simulink model "simulink_flightgear_control_trim_wind_5"  (R2023a)
settings: Solver=VariableStepAuto  StartTime=0  StopTime=inf  FixedStep=0.1  RelTol=1e-3
values from neighbouring files (symbols this model uses):
  alpha = -5:0.1:25    [Boeing747model.m]
  alpha1 = 0:0.1:14    [Boeing747model.m]
  alpha2 = -5:0.1:25    [Boeing747model.m]
  alpha3 = -5:0.1:17    [Boeing747model.m]
  beta = -15:0.1:15    [Boeing747model.m]
  CL = 0:0.01:1.4    [Boeing747model.m]
  da = 0:1:20    [Boeing747model.m]
  dr = [0 5 10 15 20 25]    [Boeing747model.m]
  EPR_ = 0:0.1:1.8    [Boeing747model.m]    (also in engine.m)
  flap = [0 10 20 25 30]    [Boeing747model.m]
  high1 = 0:10000:40000    [Boeing747model.m]
  high2 = 0:20000:40000    [Boeing747model.m]
  high3 = [0 15000 25000 35000 40000]    [Boeing747model.m]    (also in engine.m)
  high4 = [0 10000 20000 40000]    [Boeing747model.m]
  interp_result = table2array(resultTable(:,2:end))    [Boeing747model.m]
  interp_result_mach = 0:0.1:0.9    [Boeing747model.m]
  interp_result_N1 = 80:5:110    [Boeing747model.m]
  m2ft = 3.280839895013    (= 3.28083989501)    [Boeing747model.m]    (also in engine.m)
  mach = 0:0.02:0.9    [Boeing747model.m]    (also in engine.m)
  mach1 = [0 0.3 0.5 0.7 0.8 0.84 0.86 0.88 0.9]    [Boeing747model.m]
  mach2 = [0 0.3 0.5 0.7 0.8 0.9]    [Boeing747model.m]
  mach3 = [0 0.1 0.3 0.5 0.6 0.7 0.8 0.9]    [Boeing747model.m]    (also in engine.m = [0 0.1 0.3 0.5  0.7 0.8 0.9])
  mach5 = [0 0.6 0.8 0.85 0.9]    [Boeing747model.m]
  mach6 = [0 0.6 0.8 0.9]    [Boeing747model.m]
  mach7 = [0 0.3 0.5 0.74 0.8 0.84 0.86 0.88 0.9]    [Boeing747model.m]
  mach8 = [0 0.3 0.5 0.74 0.8 0.84 0.86 0.88 0.9]    [Boeing747model.m]
  model = 'simulink_flightgear_control_trim_wind_5'    [traimcode.m]
  ms2kts = 1.943844492609    (= 1.94384449261)    [Boeing747model.m]    (also in engine.m)
  powerangle_ = 0:1:130    [Boeing747model.m]    (also in engine.m)
  T = [-45 0 60 120]    [Boeing747model.m]    (also in engine.m)
  V_E = 0:20:250    [Boeing747model.m]
undefined symbols (not defined in the file or in its folder): Earth, F, ft, Light, m, MIL, Model, Newton, P3DAERO, Raphson, Receive, s, Send, Unit, WGS84, Wind
libraries: simulink_extras x115, aerolibconvert2 x16, simulink x4, aerolibfltsims x3, shared6dof x1, aerolibasang x1, aerolibtransform2 x1, aerolibatmos2 x1, aerolibobsolete x1, aerolibwind2 x1
(part 4 of 5)

== system simulink_flightgear_control_trim_wind_5/Plane/气动系数/Subsystem58/Subsystem41 ==
  In1 : Inport
  In2 : Inport  Port=2
  Radians in : Inport  Port=3
  Radians in1 : Inport  Port=4
  1-D Lookup Table79 : Lookup_n-D  NumberOfTableDimensions=1  BreakpointsForDimension1=P3DAERO.delata_CN_RL_25(1,:)  Table=P3DAERO.delata_CN_RL_25(2,:)  InternalRulePriority=Speed  RndMeth=Simplest
  1-D Lookup Table81 : Lookup_n-D  NumberOfTableDimensions=1  BreakpointsForDimension1=P3DAERO.k_delta_RL(1,:)  Table=P3DAERO.k_delta_RL(2,:)  InternalRulePriority=Speed  RndMeth=Simplest
  2-D Lookup Table15 : Lookup_n-D  BreakpointsForDimension1=high1  BreakpointsForDimension2=mach  Table=P3DAERO.delata_CN_RL_25_mach  InternalRulePriority=Speed  RndMeth=Simplest
      settings: InputPortMap=u0,u1
  Abs5 : Abs  SaturateOnIntegerOverflow=off
  Constant34 : Constant
  Constant35 : Constant  Value=-1
  Gain10 : Gain  Gain=m2ft
  Product8 : Product  Inputs=4
  Radians to Degrees22 : simulink_extras/Transformations/Radians to Degrees
  Radians to Degrees23 : simulink_extras/Transformations/Radians to Degrees
  Switch6 : Switch  SaturateOnIntegerOverflow=off  InputSameDT=off
  Out1 : Outport
  wires:
  2-D Lookup Table15/1 -> Product8/1
  Constant35/1 -> Switch6/3
  Constant34/1 -> Switch6/1
  1-D Lookup Table81/1 -> Product8/3
  Radians in1/1 -> Switch6/2, Radians to Degrees23/1
  Radians to Degrees22/1 -> 1-D Lookup Table79/1
  Abs5/1 -> 1-D Lookup Table81/1
  Gain10/1 -> 2-D Lookup Table15/1
  Switch6/1 -> Product8/4
  Radians to Degrees23/1 -> Abs5/1
  1-D Lookup Table79/1 -> Product8/2
  In2/1 -> 2-D Lookup Table15/2
  In1/1 -> Gain10/1
  Product8/1 -> Out1/1
  Radians in/1 -> Radians to Degrees22/1

== system simulink_flightgear_control_trim_wind_5/Plane/气动系数/Subsystem58/Subsystem42 ==
  note: 速度ft/s
  note: beta角速度
  Radians in : Inport
  In2 : Inport  Port=2
  In3 : Inport  Port=3
  In4 : Inport  Port=4
  In5 : Inport  Port=5
  1-D Lookup Table2 : Lookup_n-D  NumberOfTableDimensions=1  BreakpointsForDimension1=P3DAERO.dot_CN_dot_beta_dian(1,:)  Table=P3DAERO.dot_CN_dot_beta_dian(2,:)  InternalRulePriority=Speed  RndMeth=Simplest
  2-D Lookup Table4 : Lookup_n-D  BreakpointsForDimension1=high1  BreakpointsForDimension2=mach  Table=P3DAERO.dot_CN_dot_beta_dian_mach  InternalRulePriority=Speed  RndMeth=Simplest
      settings: InputPortMap=u0,u1
  Constant7 : Constant  Value=2
  Constant8 : Constant  Value=195.7
  Divide2 : Product  Inputs=**//
  Gain : Gain  Gain=-1
  Gain5 : Gain  Gain=m2ft
  Product2 : Product  Inputs=3
  Radians to Degrees : simulink_extras/Transformations/Radians to Degrees
  Scope1 : Scope
  Out1 : Outport
  wires:
  2-D Lookup Table4/1 -> Product2/2
  Divide2/1 -> Product2/3
  1-D Lookup Table2/1 -> Product2/1
  In3/1 -> 2-D Lookup Table4/2
  Constant8/1 -> Divide2/2
  Gain5/1 -> 2-D Lookup Table4/1
  Radians to Degrees/1 -> 1-D Lookup Table2/1
  Constant7/1 -> Divide2/4
  Radians in/1 -> Radians to Degrees/1
  In2/1 -> Gain5/1
  In4/1 -> Divide2/1
  Product2/1 -> Gain/1
  In5/1 -> Divide2/3
  Gain/1 -> Scope1/1, Out1/1

== system simulink_flightgear_control_trim_wind_5/Plane/气动系数/Subsystem58/Subsystem43 ==
  note: 滚转角速度
  In1 : Inport
  In2 : Inport  Port=2
  Radians in : Inport  Port=3
  In4 : Inport  Port=4
  In5 : Inport  Port=5
  2-D Lookup Table5 : Lookup_n-D  BreakpointsForDimension1=flap  BreakpointsForDimension2=alpha  Table=P3DAERO.dot_CN_dot_p  InternalRulePriority=Speed  RndMeth=Simplest
      settings: InputPortMap=u0,u1
  2-D Lookup Table6 : Lookup_n-D  BreakpointsForDimension1=mach5  BreakpointsForDimension2=alpha  Table=P3DAERO.dot_CN_dot_p_mach  InternalRulePriority=Speed  RndMeth=Simplest
      settings: InputPortMap=u0,u1
  Constant24 : Constant  Value=2
  Constant25 : Constant  Value=195.7
  Divide3 : Product  Inputs=**//
  Divide4 : Product  Inputs=**
  Gain5 : Gain  Gain=-1
  Radians to Degrees3 : simulink_extras/Transformations/Radians to Degrees
  Radians to Degrees5 : simulink_extras/Transformations/Radians to Degrees
  Scope : Scope
  Switch11 : Switch  Criteria=u2 ~= 0  Threshold=0.6  SaturateOnIntegerOverflow=off  InputSameDT=off
  Out1 : Outport
  wires:
  In2/1 -> Switch11/2, 2-D Lookup Table5/1
  Divide4/1 -> Gain5/1
  Switch11/1 -> Divide4/2
  2-D Lookup Table6/1 -> Switch11/3
  2-D Lookup Table5/1 -> Switch11/1
  Radians to Degrees5/1 -> 2-D Lookup Table5/2
  Radians in/1 -> Radians to Degrees3/1, Radians to Degrees5/1
  Radians to Degrees3/1 -> 2-D Lookup Table6/2
  Constant25/1 -> Divide3/2
  In4/1 -> 2-D Lookup Table6/1
  Divide3/1 -> Divide4/1
  Constant24/1 -> Divide3/4
  In1/1 -> Divide3/1
  In5/1 -> Divide3/3
  Gain5/1 -> Scope/1, Out1/1

== system simulink_flightgear_control_trim_wind_5/Plane/气动系数/Subsystem58/Subsystem44 ==
  u : Inport
  In2 : Inport  Port=2
  Radians in : Inport  Port=3
  In4 : Inport  Port=4
  In5 : Inport  Port=5
  In6 : Inport  Port=6
  In7 : Inport  Port=7
  2-D Lookup Table7 : Lookup_n-D  BreakpointsForDimension1=flap  BreakpointsForDimension2=alpha  Table=P3DAERO.dot_CN_dot_r25  InternalRulePriority=Speed  RndMeth=Simplest
      settings: InputPortMap=u0,u1
  2-D Lookup Table8 : Lookup_n-D  BreakpointsForDimension1=high1  BreakpointsForDimension2=mach  Table=P3DAERO.dot_CN_dot_r_mach  InternalRulePriority=Speed  RndMeth=Simplest
      settings: InputPortMap=u0,u1
  Constant13 : Constant  Value=2
  Constant14 : Constant  Value=195.7
  Divide6 : Product  Inputs=**//
  Gain7 : Gain  Gain=m2ft
  MATLAB Function2 : MATLAB Function  TreatAsAtomicUnit=on
  MATLAB Function3 : MATLAB Function  Commented=on  TreatAsAtomicUnit=on
  Product1 : Product  Inputs=4
  Radians to Degrees2 : simulink_extras/Transformations/Radians to Degrees
  Scope : Scope
  Scope1 : Scope
  Out1 : Outport
  wires:
  Constant13/1 -> Divide6/4
  2-D Lookup Table7/1 -> Product1/2
  Radians to Degrees2/1 -> 2-D Lookup Table7/2
  MATLAB Function2/1(y) -> Scope1/1, Product1/1
  2-D Lookup Table8/1 -> Product1/3
  Constant14/1 -> Divide6/2
  Gain7/1 -> 2-D Lookup Table8/1
  In2/1 -> 2-D Lookup Table7/1
  Radians in/1 -> Radians to Degrees2/1
  Divide6/1 -> Product1/4
  In5/1 -> 2-D Lookup Table8/2
  In4/1 -> Gain7/1
  In6/1 -> Divide6/1
  u/1 -> MATLAB Function2/1(u)
  In7/1 -> Divide6/3
  Product1/1 -> Scope/1, Out1/1

== system simulink_flightgear_control_trim_wind_5/Plane/气动系数/Subsystem58/Subsystem45 ==
  note: n地效修正
  In1 : Inport
  In2 : Inport  Port=2
  Radians in : Inport  Port=3
  1-D Lookup Table86 : Lookup_n-D  NumberOfTableDimensions=1  BreakpointsForDimension1=P3DAERO.k_ge(1,:)  Table=P3DAERO.k_ge(2,:)  InternalRulePriority=Speed  RndMeth=Simplest
  2-D Lookup Table9 : Lookup_n-D  BreakpointsForDimension1=flap  BreakpointsForDimension2=alpha1  Table=P3DAERO.Fn  InternalRulePriority=Speed  RndMeth=Simplest
      settings: InputPortMap=u0,u1
  Constant27 : Constant
  Gain3 : Gain  Gain=m2ft
  Product6 : Product
  Radians to Degrees7 : simulink_extras/Transformations/Radians to Degrees
  Saturation2 : Saturate  UpperLimit=14  LowerLimit=0
  Scope2 : Scope
  Sum19 : Sum
  Switch1 : Switch  Criteria=u2 > Threshold  Threshold=24  SaturateOnIntegerOverflow=off  InputSameDT=off
  Out1 : Outport
  wires:
  In2/1 -> 2-D Lookup Table9/1
  2-D Lookup Table9/1 -> Product6/2
  Gain3/1 -> 1-D Lookup Table86/1
  Radians to Degrees7/1 -> Saturation2/1
  Sum19/1 -> Switch1/3
  Saturation2/1 -> 2-D Lookup Table9/2
  1-D Lookup Table86/1 -> Product6/1, Scope2/1
  Constant27/1 -> Sum19/1, Switch1/1
  Product6/1 -> Sum19/2
  Radians in/1 -> Radians to Degrees7/1
  Switch1/1 -> Out1/1
  In1/1 -> Switch1/2, Gain3/1

== system simulink_flightgear_control_trim_wind_5/Plane/气动系数/Subsystem58/Subsystem46 ==
  In1 : Inport
  In2 : Inport  Port=2
  Radians in : Inport  Port=3
  In4 : Inport  Port=4
  Radians in1 : Inport  Port=5
  1-D Lookup Table1 : Lookup_n-D  BreakpointsForDimension1=flap  BreakpointsForDimension2=alpha  Table=P3DAERO.delta_CN_ai  InternalRulePriority=Speed  RndMeth=Simplest
      settings: InputPortMap=u0,u1
  1-D Lookup Table3 : Lookup_n-D  BreakpointsForDimension1=flap  BreakpointsForDimension2=da  Table=P3DAERO.k_delta_ai  InternalRulePriority=Speed  RndMeth=Simplest
      settings: InputPortMap=u0,u1
  1-D Lookup Table54 : Lookup_n-D  NumberOfTableDimensions=1  BreakpointsForDimension1=P3DAERO.delta_CN_ai_mach(1,:)  Table=P3DAERO.delta_CN_ai_mach(2,:)  InternalRulePriority=Speed  RndMeth=Simplest
  Constant16 : Constant
  Constant18 : Constant  Value=-1
  Constant20 : Constant  Value=2
  Product4 : Product  Inputs=3
  Product5 : Product  Inputs=4
  Radians to Degrees8 : simulink_extras/Transformations/Radians to Degrees
  Radians to Degrees9 : simulink_extras/Transformations/Radians to Degrees
  Scope4 : Scope
  Switch2 : Switch  SaturateOnIntegerOverflow=off  InputSameDT=off
  Out1 : Outport
  wires:
  1-D Lookup Table3/1 -> Product5/4
  Constant18/1 -> Switch2/3
  1-D Lookup Table54/1 -> Product5/1
  Radians to Degrees8/1 -> 1-D Lookup Table3/2
  Switch2/1 -> Product4/3
  1-D Lookup Table1/1 -> Product5/2
  Radians to Degrees9/1 -> 1-D Lookup Table1/2
  Radians in1/1 -> Switch2/2, Radians to Degrees8/1
  Constant16/1 -> Switch2/1
  Constant20/1 -> Product4/1
  Product5/1 -> Product4/2, Scope4/1
  In2/1 -> 1-D Lookup Table3/1, 1-D Lookup Table1/1
  In4/1 -> Product5/3
  Radians in/1 -> Radians to Degrees9/1
  Product4/1 -> Out1/1
  In1/1 -> 1-D Lookup Table54/1

== system simulink_flightgear_control_trim_wind_5/Plane/气动系数/Subsystem58/Subsystem47 ==
  note: 15down
  note: 25up
  In1 : Inport
  Radians in : Inport  Port=2
  In3 : Inport  Port=3
  Radians in1 : Inport  Port=4
  1-D Lookup Table60 : Lookup_n-D  NumberOfTableDimensions=1  BreakpointsForDimension1=P3DAERO.k_delata_Ao_down(1,:)  Table=P3DAERO.k_delata_Ao_down(2,:)  InternalRulePriority=Speed  RndMeth=Simplest
  1-D Lookup Table61 : Lookup_n-D  NumberOfTableDimensions=1  BreakpointsForDimension1=P3DAERO.k_delata_Ao_up(1,:)  Table=P3DAERO.k_delata_Ao_up(2,:)  InternalRulePriority=Speed  RndMeth=Simplest
  2-D Lookup Table10 : Lookup_n-D  BreakpointsForDimension1=flap  BreakpointsForDimension2=alpha  Table=P3DAERO.delata_CN_Ao_15down  InternalRulePriority=Speed  RndMeth=Simplest
      settings: InputPortMap=u0,u1
  2-D Lookup Table11 : Lookup_n-D  BreakpointsForDimension1=flap  BreakpointsForDimension2=alpha  Table=P3DAERO.delata_CN_Ao_25up  InternalRulePriority=Speed  RndMeth=Simplest
      settings: InputPortMap=u0,u1
  Abs3 : Abs  SaturateOnIntegerOverflow=off
  Abs4 : Abs  SaturateOnIntegerOverflow=off
  Product13 : Product  Inputs=3
  Radians to Degrees{10,15..17} (4 alike) : simulink_extras/Transformations/Radians to Degrees
  Scope34 : Scope
  Scope37 : Scope
  Scope38 : Scope
  Switch7 : Switch  SaturateOnIntegerOverflow=off  InputSameDT=off
  Switch8 : Switch  SaturateOnIntegerOverflow=off  InputSameDT=off
  Out1 : Outport
  wires:
  Switch7/1 -> Product13/2, Scope34/1
  Radians to Degrees16/1 -> 2-D Lookup Table11/2
  Radians in/1 -> Radians to Degrees17/1, Switch8/2, Radians to Degrees15/1, Switch7/2
  2-D Lookup Table11/1 -> Switch8/3
  Abs3/1 -> 1-D Lookup Table60/1
  Switch8/1 -> Product13/3, Scope37/1
  Radians to Degrees15/1 -> Abs3/1
  In3/1 -> 2-D Lookup Table11/1, 2-D Lookup Table10/1
  1-D Lookup Table60/1 -> Switch7/1
  2-D Lookup Table10/1 -> Switch8/1
  Radians to Degrees10/1 -> 2-D Lookup Table10/2
  Abs4/1 -> 1-D Lookup Table61/1
  Radians to Degrees17/1 -> Abs4/1
  1-D Lookup Table61/1 -> Switch7/3
  Product13/1 -> Out1/1, Scope38/1
  Radians in1/1 -> Radians to Degrees16/1, Radians to Degrees10/1
  In1/1 -> Product13/1

== system simulink_flightgear_control_trim_wind_5/Plane/气动系数/Subsystem58/Subsystem48 ==
  note: 15down
  note: 25up
  In1 : Inport
  Radians in : Inport  Port=2
  In3 : Inport  Port=3
  Radians in1 : Inport  Port=4
  1-D Lookup Table72 : Lookup_n-D  NumberOfTableDimensions=1  BreakpointsForDimension1=P3DAERO.k_delata_Ao_down(1,:)  Table=P3DAERO.k_delata_Ao_down(2,:)  InternalRulePriority=Speed  RndMeth=Simplest
  1-D Lookup Table73 : Lookup_n-D  NumberOfTableDimensions=1  BreakpointsForDimension1=P3DAERO.k_delata_Ao_up(1,:)  Table=P3DAERO.k_delata_Ao_up(2,:)  InternalRulePriority=Speed  RndMeth=Simplest
  2-D Lookup Table12 : Lookup_n-D  BreakpointsForDimension1=flap  BreakpointsForDimension2=alpha  Table=P3DAERO.delata_CN_Ao_15down  InternalRulePriority=Speed  RndMeth=Simplest
      settings: InputPortMap=u0,u1
  2-D Lookup Table13 : Lookup_n-D  BreakpointsForDimension1=flap  BreakpointsForDimension2=alpha  Table=P3DAERO.delata_CN_Ao_25up  InternalRulePriority=Speed  RndMeth=Simplest
      settings: InputPortMap=u0,u1
  Abs1 : Abs  SaturateOnIntegerOverflow=off
  Abs2 : Abs  SaturateOnIntegerOverflow=off
  Product14 : Product  Inputs=3
  Radians to Degrees{11..14} (4 alike) : simulink_extras/Transformations/Radians to Degrees
  Scope39 : Scope
  Scope43 : Scope
  Switch3 : Switch  SaturateOnIntegerOverflow=off  InputSameDT=off
  Switch9 : Switch  SaturateOnIntegerOverflow=off  InputSameDT=off
  Out1 : Outport
  wires:
  Switch3/1 -> Product14/3
  Radians to Degrees12/1 -> Abs1/1
  In3/1 -> 2-D Lookup Table13/1, 2-D Lookup Table12/1
  1-D Lookup Table72/1 -> Switch9/1
  Radians in1/1 -> Radians to Degrees14/1, Radians to Degrees11/1
  2-D Lookup Table13/1 -> Switch3/3
  Abs1/1 -> 1-D Lookup Table72/1
  Switch9/1 -> Product14/2, Scope39/1
  Radians to Degrees13/1 -> Abs2/1
  Radians to Degrees11/1 -> 2-D Lookup Table12/2
  Radians to Degrees14/1 -> 2-D Lookup Table13/2
  Product14/1 -> Out1/1, Scope43/1
  2-D Lookup Table12/1 -> Switch3/1
  Abs2/1 -> 1-D Lookup Table73/1
  1-D Lookup Table73/1 -> Switch9/3
  Radians in/1 -> Radians to Degrees13/1, Switch3/2, Radians to Degrees12/1, Switch9/2
  In1/1 -> Product14/1

== system simulink_flightgear_control_trim_wind_5/Plane/气动系数/Subsystem58/Subsystem49 ==
  note: Y beta地效修正
  In1 : Inport
  In2 : Inport  Port=2
  Radians in : Inport  Port=3
  1-D Lookup Table97 : Lookup_n-D  NumberOfTableDimensions=1  BreakpointsForDimension1=P3DAERO.k_ge(1,:)  Table=P3DAERO.k_ge(2,:)  InternalRulePriority=Speed  RndMeth=Simplest
  2-D Lookup Table2 : Lookup_n-D  BreakpointsForDimension1=flap  BreakpointsForDimension2=alpha1  Table=P3DAERO.Fc_beta  InternalRulePriority=Speed  RndMeth=Simplest
      settings: InputPortMap=u0,u1
  Constant : Constant  Value=4.58
  Constant21 : Constant
  Gain14 : Gain  Gain=m2ft
  Product16 : Product
  Radians to Degrees1 : simulink_extras/Transformations/Radians to Degrees
  Saturation2 : Saturate  UpperLimit=14  LowerLimit=0
  Scope31 : Scope
  Scope48 : Scope
  Sum : Sum  Inputs=|+-
  Sum11 : Sum
  Switch5 : Switch  Criteria=u2 > Threshold  Threshold=24  SaturateOnIntegerOverflow=off  InputSameDT=off
  Out1 : Outport
  wires:
  Gain14/1 -> 1-D Lookup Table97/1
  Switch5/1 -> Out1/1, Scope31/1
  Saturation2/1 -> 2-D Lookup Table2/2
  Radians to Degrees1/1 -> Saturation2/1
  Product16/1 -> Sum11/2
  Constant21/1 -> Sum11/1, Switch5/1
  1-D Lookup Table97/1 -> Scope48/1, Product16/1
  Sum11/1 -> Switch5/3
  2-D Lookup Table2/1 -> Product16/2
  In2/1 -> 2-D Lookup Table2/1
  Radians in/1 -> Radians to Degrees1/1
  Constant/1 -> Sum/2
  In1/1 -> Sum/1
  Sum/1 -> Switch5/2, Gain14/1

== system simulink_flightgear_control_trim_wind_5/Plane/气动系数/Subsystem58/Subsystem5 ==
  note: 迎角角速度rad/s
  note: 速度ft/s
  note: dot_CL_dot_alpha_dian
  note: 平均气动弦长ft
  In1 : Inport
  In2 : Inport  Port=2
  In3 : Inport  Port=3
  1-D Lookup Table1 : Lookup_n-D  NumberOfTableDimensions=1  BreakpointsForDimension1=mach  Table=P3DAERO.dot_CL_dot_alpha_dian  InternalRulePriority=Speed  RndMeth=Simplest
  Constant7 : Constant  Value=2
  Constant9 : Constant  Value=27.3
  Divide : Product  Inputs=**//
  Gain8 : Gain
  Product2 : Product
  Scope5 : Scope
  Scope8 : Scope
  Scope9 : Scope
  Out1 : Outport
  wires:
  In2/1 -> 1-D Lookup Table1/1
  Gain8/1 -> Out1/1, Scope9/1
  Constant9/1 -> Divide/2
  Constant7/1 -> Divide/4
  Product2/1 -> Gain8/1
  Divide/1 -> Product2/2, Scope5/1
  1-D Lookup Table1/1 -> Product2/1, Scope8/1
  In1/1 -> Divide/1
  In3/1 -> Divide/3

== system simulink_flightgear_control_trim_wind_5/Plane/气动系数/Subsystem58/Subsystem50 ==
  In1 : Inport
  Radians in : Inport  Port=2
  In3 : Inport  Port=3
  In4 : Inport  Port=4
  2-D Lookup Table : Lookup_n-D  BreakpointsForDimension1=flap  BreakpointsForDimension2=alpha  Table=P3DAERO.dot_CC_dot_beta  InternalRulePriority=Speed  RndMeth=Simplest
      settings: InputPortMap=u0,u1
  2-D Lookup Table1 : Lookup_n-D  BreakpointsForDimension1=high1  BreakpointsForDimension2=mach  Table=P3DAERO.dot_CC_dot_beta_mach  InternalRulePriority=Speed  RndMeth=Simplest
      settings: InputPortMap=u0,u1
  Gain3 : Gain  Gain=m2ft
  Product : Product
  Radians to Degrees4 : simulink_extras/Transformations/Radians to Degrees
  Out1 : Outport
  wires:
  2-D Lookup Table/1 -> Product/1
  Gain3/1 -> 2-D Lookup Table1/1
  Radians to Degrees4/1 -> 2-D Lookup Table/2
  2-D Lookup Table1/1 -> Product/2
  In3/1 -> Gain3/1
  In4/1 -> 2-D Lookup Table1/2
  Radians in/1 -> Radians to Degrees4/1
  In1/1 -> 2-D Lookup Table/1
  Product/1 -> Out1/1

== system simulink_flightgear_control_trim_wind_5/Plane/气动系数/Subsystem58/Subsystem51 ==
  note: 滚转角速度
  note: bft
  note: 速度ft/s
  In1 : Inport
  In2 : Inport  Port=2
  In3 : Inport  Port=3
  Radians in : Inport  Port=4
  In5 : Inport  Port=5
  2-D Lookup Table3 : Lookup_n-D  BreakpointsForDimension1=flap  BreakpointsForDimension2=alpha  Table=P3DAERO.dot_CC_dot_p  InternalRulePriority=Speed  RndMeth=Simplest
      settings: InputPortMap=u0,u1
  2-D Lookup Table4 : Lookup_n-D  BreakpointsForDimension1=mach6  BreakpointsForDimension2=alpha  Table=P3DAERO.dot_CC_dot_p_mach  InternalRulePriority=Speed  RndMeth=Simplest
      settings: InputPortMap=u0,u1
  Constant10 : Constant  Value=2
  Constant12 : Constant  Value=195.7
  Divide1 : Product  Inputs=**//
  Divide3 : Product  Inputs=**
  Gain : Gain  Gain=-1
  Radians to Degrees5 : simulink_extras/Transformations/Radians to Degrees
  Radians to Degrees6 : simulink_extras/Transformations/Radians to Degrees
  Scope : Scope
  Switch3 : Switch  Criteria=u2 ~= 0  Threshold=0.6  SaturateOnIntegerOverflow=off  InputSameDT=off
  Out1 : Outport
  wires:
  Radians in/1 -> Radians to Degrees5/1, Radians to Degrees6/1
  In2/1 -> 2-D Lookup Table4/1
  In1/1 -> Divide1/1
  Divide1/1 -> Divide3/1
  Switch3/1 -> Divide3/2
  Radians to Degrees6/1 -> 2-D Lookup Table3/2
  2-D Lookup Table3/1 -> Switch3/1
  Constant12/1 -> Divide1/2
  Radians to Degrees5/1 -> 2-D Lookup Table4/2
  In3/1 -> Switch3/2, 2-D Lookup Table3/1
  Constant10/1 -> Divide1/4
  2-D Lookup Table4/1 -> Switch3/3
  Divide3/1 -> Scope/1, Gain/1
  In5/1 -> Divide1/3
  Gain/1 -> Out1/1

== system simulink_flightgear_control_trim_wind_5/Plane/气动系数/Subsystem58/Subsystem52 ==
  note: 速度ft/s
  note: 偏航角速度
  In1 : Inport
  Radians in : Inport  Port=2
  In3 : Inport  Port=3
  In4 : Inport  Port=4
  In5 : Inport  Port=5
  In6 : Inport  Port=6
  2-D Lookup Table5 : Lookup_n-D  BreakpointsForDimension1=flap  BreakpointsForDimension2=alpha  Table=P3DAERO.dot_CC_dot_r  InternalRulePriority=Speed  RndMeth=Simplest
      settings: InputPortMap=u0,u1
  2-D Lookup Table6 : Lookup_n-D  BreakpointsForDimension1=high4  BreakpointsForDimension2=mach  Table=P3DAERO.dot_CC_dot_r_mach  InternalRulePriority=Speed  RndMeth=Simplest
      settings: InputPortMap=u0,u1
  Constant7 : Constant  Value=2
  Constant8 : Constant  Value=195.7
  Divide2 : Product  Inputs=**//
  Gain4 : Gain  Gain=m2ft
  Product2 : Product  Inputs=3
  Radians to Degrees7 : simulink_extras/Transformations/Radians to Degrees
  Scope : Scope
  Out1 : Outport
  wires:
  2-D Lookup Table5/1 -> Product2/1
  In4/1 -> 2-D Lookup Table6/2
  Divide2/1 -> Product2/3
  Gain4/1 -> 2-D Lookup Table6/1
  Constant8/1 -> Divide2/2
  Radians to Degrees7/1 -> 2-D Lookup Table5/2
  2-D Lookup Table6/1 -> Product2/2
  Constant7/1 -> Divide2/4
  Radians in/1 -> Radians to Degrees7/1
  In1/1 -> 2-D Lookup Table5/1
  In3/1 -> Gain4/1
  In5/1 -> Divide2/1
  In6/1 -> Divide2/3
  Product2/1 -> Out1/1, Scope/1

== system simulink_flightgear_control_trim_wind_5/Plane/气动系数/Subsystem58/Subsystem53 ==
  In1 : Inport
  In2 : Inport  Port=2
  Radians in : Inport  Port=3
  Radians in1 : Inport  Port=4
  1-D Lookup Table101 : Lookup_n-D  NumberOfTableDimensions=1  BreakpointsForDimension1=P3DAERO.delta_CC_25_RU(1,:)  Table=P3DAERO.delta_CC_25_RU(2,:)  InternalRulePriority=Speed  RndMeth=Simplest
  1-D Lookup Table102 : Lookup_n-D  NumberOfTableDimensions=1  BreakpointsForDimension1=P3DAERO.k_delta_RU(1,:)  Table=P3DAERO.k_delta_RU(2,:)  InternalRulePriority=Speed  RndMeth=Simplest
  2-D Lookup Table7 : Lookup_n-D  BreakpointsForDimension1=high1  BreakpointsForDimension2=mach  Table=P3DAERO.delta_CC_25_RU_mach  InternalRulePriority=Speed  RndMeth=Simplest
      settings: InputPortMap=u0,u1
  Abs : Abs  SaturateOnIntegerOverflow=off
  Constant32 : Constant
  Constant33 : Constant  Value=-1
  Gain5 : Gain  Gain=m2ft
  Product7 : Product  Inputs=4
  Radians to Degrees20 : simulink_extras/Transformations/Radians to Degrees
  Radians to Degrees21 : simulink_extras/Transformations/Radians to Degrees
  Scope : Scope
  Switch12 : Switch  SaturateOnIntegerOverflow=off  InputSameDT=off
  Out1 : Outport
  wires:
  Radians to Degrees21/1 -> Abs/1
  1-D Lookup Table101/1 -> Product7/2
  Radians in1/1 -> Switch12/2, Radians to Degrees21/1
  Gain5/1 -> 2-D Lookup Table7/1
  Constant33/1 -> Switch12/3
  Radians to Degrees20/1 -> 1-D Lookup Table101/1
  Abs/1 -> 1-D Lookup Table102/1
  Switch12/1 -> Product7/4
  Constant32/1 -> Switch12/1
  1-D Lookup Table102/1 -> Product7/3
  2-D Lookup Table7/1 -> Product7/1
  In1/1 -> Gain5/1
  In2/1 -> 2-D Lookup Table7/2
  Radians in/1 -> Radians to Degrees20/1
  Product7/1 -> Scope/1, Out1/1

== system simulink_flightgear_control_trim_wind_5/Plane/气动系数/Subsystem58/Subsystem54 ==
  In1 : Inport
  In2 : Inport  Port=2
  Radians in : Inport  Port=3
  Radians in1 : Inport  Port=4
  1-D Lookup Table79 : Lookup_n-D  NumberOfTableDimensions=1  BreakpointsForDimension1=P3DAERO.delta_CC_25_RL(1,:)  Table=P3DAERO.delta_CC_25_RL(2,:)  InternalRulePriority=Speed  RndMeth=Simplest
  1-D Lookup Table81 : Lookup_n-D  NumberOfTableDimensions=1  BreakpointsForDimension1=P3DAERO.k_delta_RL(1,:)  Table=P3DAERO.k_delta_RL(2,:)  InternalRulePriority=Speed  RndMeth=Simplest
  2-D Lookup Table8 : Lookup_n-D  BreakpointsForDimension1=high1  BreakpointsForDimension2=mach  Table=P3DAERO.delta_CC_25_RL_mach  InternalRulePriority=Speed  RndMeth=Simplest
      settings: InputPortMap=u0,u1
  Abs5 : Abs  SaturateOnIntegerOverflow=off
  Constant34 : Constant
  Constant35 : Constant  Value=-1
  Gain7 : Gain  Gain=m2ft
  Product8 : Product  Inputs=4
  Radians to Degrees22 : simulink_extras/Transformations/Radians to Degrees
  Radians to Degrees23 : simulink_extras/Transformations/Radians to Degrees
  Switch6 : Switch  SaturateOnIntegerOverflow=off  InputSameDT=off
  Out1 : Outport
  wires:
  Abs5/1 -> 1-D Lookup Table81/1
  2-D Lookup Table8/1 -> Product8/1
  Gain7/1 -> 2-D Lookup Table8/1
  Radians in1/1 -> Switch6/2, Radians to Degrees23/1
  1-D Lookup Table79/1 -> Product8/2
  In1/1 -> Gain7/1
  Constant34/1 -> Switch6/1
  Constant35/1 -> Switch6/3
  Radians to Degrees22/1 -> 1-D Lookup Table79/1
  Switch6/1 -> Product8/4
  Radians to Degrees23/1 -> Abs5/1
  Radians in/1 -> Radians to Degrees22/1
  1-D Lookup Table81/1 -> Product8/3
  In2/1 -> 2-D Lookup Table8/2
  Product8/1 -> Out1/1

== system simulink_flightgear_control_trim_wind_5/Plane/气动系数/Subsystem58/Subsystem55 ==
  In1 : Inport
  Radians in : Inport  Port=2
  Gain : Gain  Gain=-0.002
  Product15 : Product
  Radians to Degrees2 : simulink_extras/Transformations/Radians to Degrees
  Scope47 : Scope
  Out1 : Outport
  wires:
  Product15/1 -> Out1/1, Scope47/1
  Radians to Degrees2/1 -> Gain/1
  Gain/1 -> Product15/2
  In1/1 -> Product15/1
  Radians in/1 -> Radians to Degrees2/1

== system simulink_flightgear_control_trim_wind_5/Plane/气动系数/Subsystem58/Subsystem56 ==
  note: 15down
  note: 25up
  In1 : Inport
  Radians in : Inport  Port=2
  In3 : Inport  Port=3
  Radians in1 : Inport  Port=4
  In5 : Inport  Port=5
  1-D Lookup Table60 : Lookup_n-D  NumberOfTableDimensions=1  BreakpointsForDimension1=P3DAERO.k_delata_Ao_down(1,:)  Table=P3DAERO.k_delata_Ao_down(2,:)  InternalRulePriority=Speed  RndMeth=Simplest
  1-D Lookup Table61 : Lookup_n-D  NumberOfTableDimensions=1  BreakpointsForDimension1=P3DAERO.k_delata_Ao_up(1,:)  Table=P3DAERO.k_delata_Ao_up(2,:)  InternalRulePriority=Speed  RndMeth=Simplest
  1-D Lookup Table99 : Lookup_n-D  NumberOfTableDimensions=1  BreakpointsForDimension1=V_E  Table=P3DAERO.Cl_Ao_aeroelastic  InternalRulePriority=Speed  RndMeth=Simplest
  2-D Lookup Table13 : Lookup_n-D  BreakpointsForDimension1=flap  BreakpointsForDimension2=alpha  Table=P3DAERO.delata_Cl_Ao_15down  InternalRulePriority=Speed  RndMeth=Simplest
      settings: InputPortMap=u0,u1
  2-D Lookup Table14 : Lookup_n-D  BreakpointsForDimension1=flap  BreakpointsForDimension2=alpha  Table=P3DAERO.delata_Cl_Ao_25up  InternalRulePriority=Speed  RndMeth=Simplest
      settings: InputPortMap=u0,u1
  Abs3 : Abs  SaturateOnIntegerOverflow=off
  Abs4 : Abs  SaturateOnIntegerOverflow=off
  Gain : Gain  Gain=-1
  Product13 : Product  Inputs=4
  Radians to Degrees{8,10,15,17} (4 alike) : simulink_extras/Transformations/Radians to Degrees
  Scope1 : Scope
  Scope34 : Scope
  Scope38 : Scope
  Switch7 : Switch  SaturateOnIntegerOverflow=off  InputSameDT=off
  Switch8 : Switch  SaturateOnIntegerOverflow=off  InputSameDT=off
  Out1 : Outport
  wires:
  1-D Lookup Table99/1 -> Product13/4
  Radians in/1 -> Switch8/2, Radians to Degrees17/1, Radians to Degrees15/1, Switch7/2
  1-D Lookup Table60/1 -> Switch7/1
  In3/1 -> 2-D Lookup Table14/1, 2-D Lookup Table13/1
  Product13/1 -> Out1/1, Scope38/1
  Abs4/1 -> 1-D Lookup Table61/1
  Radians to Degrees15/1 -> Abs3/1
  2-D Lookup Table14/1 -> Switch8/3
  Radians to Degrees8/1 -> 2-D Lookup Table13/2
  Radians in1/1 -> Radians to Degrees10/1, Radians to Degrees8/1
  1-D Lookup Table61/1 -> Switch7/3
  Switch8/1 -> Gain/1
  2-D Lookup Table13/1 -> Switch8/1
  Abs3/1 -> 1-D Lookup Table60/1
  In5/1 -> 1-D Lookup Table99/1
  Radians to Degrees17/1 -> Abs4/1
  Switch7/1 -> Product13/2, Scope34/1
  Radians to Degrees10/1 -> 2-D Lookup Table14/2
  In1/1 -> Product13/1
  Gain/1 -> Scope1/1, Product13/3

== system simulink_flightgear_control_trim_wind_5/Plane/气动系数/Subsystem58/Subsystem57 ==
  note: 25up
  note: 15down
  In1 : Inport
  Radians in : Inport  Port=2
  In3 : Inport  Port=3
  Radians in1 : Inport  Port=4
  In5 : Inport  Port=5
  1-D Lookup Table100 : Lookup_n-D  NumberOfTableDimensions=1  BreakpointsForDimension1=V_E  Table=P3DAERO.Cl_Ao_aeroelastic  InternalRulePriority=Speed  RndMeth=Simplest
  1-D Lookup Table72 : Lookup_n-D  NumberOfTableDimensions=1  BreakpointsForDimension1=P3DAERO.k_delata_Ao_down(1,:)  Table=P3DAERO.k_delata_Ao_down(2,:)  InternalRulePriority=Speed  RndMeth=Simplest
  1-D Lookup Table73 : Lookup_n-D  NumberOfTableDimensions=1  BreakpointsForDimension1=P3DAERO.k_delata_Ao_up(1,:)  Table=P3DAERO.k_delata_Ao_up(2,:)  InternalRulePriority=Speed  RndMeth=Simplest
  2-D Lookup Table15 : Lookup_n-D  BreakpointsForDimension1=flap  BreakpointsForDimension2=alpha  Table=P3DAERO.delata_Cl_Ao_15down  InternalRulePriority=Speed  RndMeth=Simplest
      settings: InputPortMap=u0,u1
  2-D Lookup Table16 : Lookup_n-D  BreakpointsForDimension1=flap  BreakpointsForDimension2=alpha  Table=P3DAERO.delata_Cl_Ao_25up  InternalRulePriority=Speed  RndMeth=Simplest
      settings: InputPortMap=u0,u1
  Abs1 : Abs  SaturateOnIntegerOverflow=off
  Abs2 : Abs  SaturateOnIntegerOverflow=off
  Product14 : Product  Inputs=4
  Radians to Degrees{11..14} (4 alike) : simulink_extras/Transformations/Radians to Degrees
  Scope39 : Scope
  Scope42 : Scope
  Scope43 : Scope
  Switch10 : Switch  SaturateOnIntegerOverflow=off  InputSameDT=off
  Switch9 : Switch  SaturateOnIntegerOverflow=off  InputSameDT=off
  Out1 : Outport
  wires:
  Abs2/1 -> 1-D Lookup Table73/1
  Radians to Degrees13/1 -> Abs2/1
  Switch10/1 -> Product14/3, Scope42/1
  In3/1 -> 2-D Lookup Table16/1, 2-D Lookup Table15/1
  Abs1/1 -> 1-D Lookup Table72/1
  Radians to Degrees14/1 -> 2-D Lookup Table15/2
  Radians to Degrees12/1 -> Abs1/1
  1-D Lookup Table100/1 -> Product14/4
  1-D Lookup Table72/1 -> Switch9/1
  Switch9/1 -> Product14/2, Scope39/1
  Radians in/1 -> Switch10/2, Radians to Degrees13/1, Radians to Degrees12/1, Switch9/2
  1-D Lookup Table73/1 -> Switch9/3
  In5/1 -> 1-D Lookup Table100/1
  Radians in1/1 -> Radians to Degrees11/1, Radians to Degrees14/1
  2-D Lookup Table16/1 -> Switch10/3
  2-D Lookup Table15/1 -> Switch10/1
  Radians to Degrees11/1 -> 2-D Lookup Table16/2
  In1/1 -> Product14/1
  Product14/1 -> Scope43/1, Out1/1

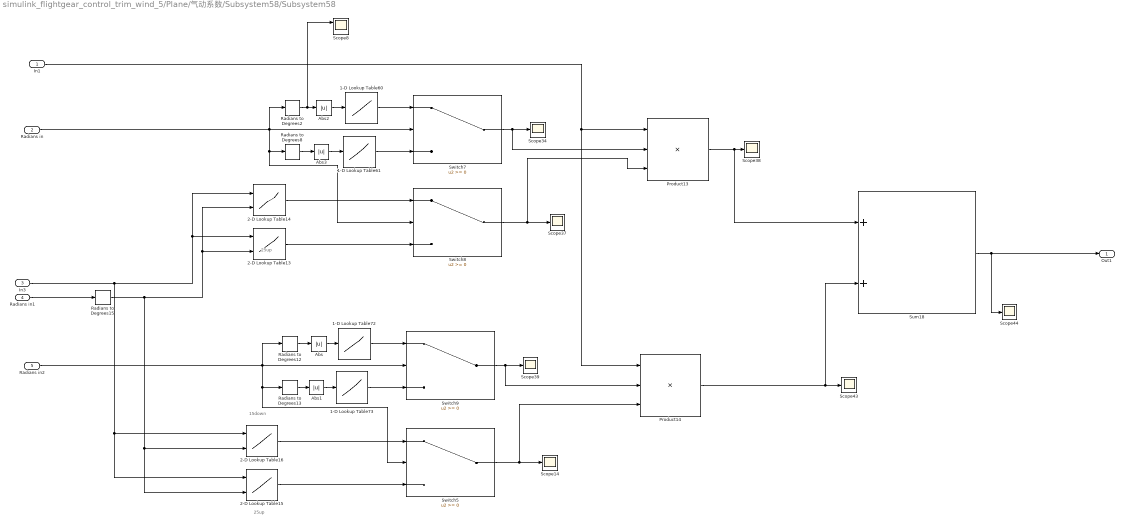
== system simulink_flightgear_control_trim_wind_5/Plane/气动系数/Subsystem58/Subsystem58 ==
  note: 25up
  note: 15down
  note: 25up
  In1 : Inport
  Radians in : Inport  Port=2
  In3 : Inport  Port=3
  Radians in1 : Inport  Port=4
  Radians in2 : Inport  Port=5
  1-D Lookup Table60 : Lookup_n-D  NumberOfTableDimensions=1  BreakpointsForDimension1=P3DAERO.k_delata_Ao_down(1,:)  Table=P3DAERO.k_delata_Ao_down(2,:)  InternalRulePriority=Speed  RndMeth=Simplest
  1-D Lookup Table61 : Lookup_n-D  NumberOfTableDimensions=1  BreakpointsForDimension1=P3DAERO.k_delata_Ao_up(1,:)  Table=P3DAERO.k_delata_Ao_up(2,:)  InternalRulePriority=Speed  RndMeth=Simplest
  1-D Lookup Table72 : Lookup_n-D  NumberOfTableDimensions=1  BreakpointsForDimension1=P3DAERO.k_delata_Ao_down(1,:)  Table=P3DAERO.k_delata_Ao_down(2,:)  InternalRulePriority=Speed  RndMeth=Simplest
  1-D Lookup Table73 : Lookup_n-D  NumberOfTableDimensions=1  BreakpointsForDimension1=P3DAERO.k_delata_Ao_up(1,:)  Table=P3DAERO.k_delata_Ao_up(2,:)  InternalRulePriority=Speed  RndMeth=Simplest
  2-D Lookup Table13 : Lookup_n-D  BreakpointsForDimension1=flap  BreakpointsForDimension2=alpha  Table=P3DAERO.delata_CL_Ao_25up  InternalRulePriority=Speed  RndMeth=Simplest
      settings: InputPortMap=u0,u1
  2-D Lookup Table14 : Lookup_n-D  BreakpointsForDimension1=flap  BreakpointsForDimension2=alpha  Table=P3DAERO.delata_CL_Ao_15down  InternalRulePriority=Speed  RndMeth=Simplest
      settings: InputPortMap=u0,u1
  2-D Lookup Table15 : Lookup_n-D  BreakpointsForDimension1=flap  BreakpointsForDimension2=alpha  Table=P3DAERO.delata_CL_Ao_25up  InternalRulePriority=Speed  RndMeth=Simplest
      settings: InputPortMap=u0,u1
  2-D Lookup Table16 : Lookup_n-D  BreakpointsForDimension1=flap  BreakpointsForDimension2=alpha  Table=P3DAERO.delata_CL_Ao_15down  InternalRulePriority=Speed  RndMeth=Simplest
      settings: InputPortMap=u0,u1
  Abs{,1..3} (4 alike) : Abs  SaturateOnIntegerOverflow=off
  Product13 : Product  Inputs=3
  Product14 : Product  Inputs=3
  Radians to Degrees{2,8,12..13,15} (5 alike) : simulink_extras/Transformations/Radians to Degrees
  Scope{14,34,37..39,43..44} (7 alike) : Scope
  Scope8 : Scope  NumInputPorts=2
  Sum18 : Sum
  Switch{5,7..9} (4 alike) : Switch  SaturateOnIntegerOverflow=off  InputSameDT=off
  Out1 : Outport
  wires:
  Radians to Degrees12/1 -> Abs/1
  Product13/1 -> Sum18/1, Scope38/1
  Switch5/1 -> Product14/3, Scope14/1
  Abs/1 -> 1-D Lookup Table72/1
  Switch8/1 -> Scope37/1, Product13/3
  Radians to Degrees15/1 -> 2-D Lookup Table15/2, 2-D Lookup Table16/2, 2-D Lookup Table14/2, 2-D Lookup Table13/2
  Radians in2/1 -> Switch5/2, Radians to Degrees13/1, Radians to Degrees12/1, Switch9/2
  Radians to Degrees13/1 -> Abs1/1
  Product14/1 -> Scope43/1, Sum18/2
  Sum18/1 -> Out1/1, Scope44/1
  Abs3/1 -> 1-D Lookup Table61/1
  2-D Lookup Table16/1 -> Switch5/1
  Radians to Degrees2/1 -> Scope8/1, Abs2/1
  1-D Lookup Table73/1 -> Switch9/3
  In1/1 -> Product14/1, Product13/1
  2-D Lookup Table13/1 -> Switch8/3
  1-D Lookup Table72/1 -> Switch9/1
  2-D Lookup Table14/1 -> Switch8/1
  1-D Lookup Table61/1 -> Switch7/3
  In3/1 -> 2-D Lookup Table15/1, 2-D Lookup Table16/1, 2-D Lookup Table14/1, 2-D Lookup Table13/1
  Switch7/1 -> Product13/2, Scope34/1
  Radians in1/1 -> Radians to Degrees15/1
  2-D Lookup Table15/1 -> Switch5/3
  Radians to Degrees8/1 -> Abs3/1
  Switch9/1 -> Product14/2, Scope39/1
  1-D Lookup Table60/1 -> Switch7/1
  Abs1/1 -> 1-D Lookup Table73/1
  Radians in/1 -> Radians to Degrees8/1, Switch8/2, Radians to Degrees2/1, Switch7/2
  Abs2/1 -> 1-D Lookup Table60/1

== system simulink_flightgear_control_trim_wind_5/Plane/气动系数/Subsystem58/Subsystem59 ==
  In1 : Inport
  In2 : Inport  Port=2
  Radians in : Inport  Port=3
  In4 : Inport  Port=4
  1-D Lookup Table101 : Lookup_n-D  NumberOfTableDimensions=1  BreakpointsForDimension1=P3DAERO.delta_Cl_RU_25(1,:)  Table=P3DAERO.delta_Cl_RU_25(2,:)  InternalRulePriority=Speed  RndMeth=Simplest
  1-D Lookup Table102 : Lookup_n-D  NumberOfTableDimensions=1  BreakpointsForDimension1=P3DAERO.k_delta_RU(1,:)  Table=P3DAERO.k_delta_RU(2,:)  InternalRulePriority=Speed  RndMeth=Simplest
  2-D Lookup Table13 : Lookup_n-D  BreakpointsForDimension1=high1  BreakpointsForDimension2=mach  Table=P3DAERO.delta_Cl_RU_mach  InternalRulePriority=Speed  RndMeth=Simplest
      settings: InputPortMap=u0,u1
  Abs : Abs  SaturateOnIntegerOverflow=off
  Constant32 : Constant
  Constant33 : Constant  Value=-1
  Gain5 : Gain  Gain=m2ft
  Product7 : Product  Inputs=4
  Radians to Degrees20 : simulink_extras/Transformations/Radians to Degrees
  Radians to Degrees21 : simulink_extras/Transformations/Radians to Degrees
  Switch12 : Switch  SaturateOnIntegerOverflow=off  InputSameDT=off
  Out1 : Outport
  wires:
  Abs/1 -> 1-D Lookup Table102/1
  Constant33/1 -> Switch12/3
  In4/1 -> Switch12/2, Radians to Degrees21/1
  Gain5/1 -> 2-D Lookup Table13/1
  In1/1 -> Gain5/1
  Radians to Degrees20/1 -> 1-D Lookup Table101/1
  Radians to Degrees21/1 -> Abs/1
  2-D Lookup Table13/1 -> Product7/1
  1-D Lookup Table101/1 -> Product7/2
  Switch12/1 -> Product7/4
  1-D Lookup Table102/1 -> Product7/3
  Constant32/1 -> Switch12/1
  In2/1 -> 2-D Lookup Table13/2
  Radians in/1 -> Radians to Degrees20/1
  Product7/1 -> Out1/1

== system simulink_flightgear_control_trim_wind_5/Plane/气动系数/Subsystem58/Subsystem6 ==
  note: 俯仰角速度rad/s
  note: dot_CL_dot_q
  note: 平均气动弦长ft
  u : Inport
  In2 : Inport  Port=2
  In3 : Inport  Port=3
  In4 : Inport  Port=4
  In5 : Inport  Port=5
  2-D Lookup Table5 : Lookup_n-D  BreakpointsForDimension1=high2  BreakpointsForDimension2=mach  Table=P3DAERO.dot_CL_dot_q  InternalRulePriority=Speed  RndMeth=Simplest
      settings: InputPortMap=u0,u1
  Constant10 : Constant  Value=27.3
  Constant12 : Constant  Value=2
  Divide1 : Product  Inputs=**//
  MATLAB Function15 : MATLAB Function  TreatAsAtomicUnit=on
  Product3 : Product  Inputs=3
  Scope10 : Scope
  Scope11 : Scope
  Scope13 : Scope
  Velocity Conversion : aerolibconvert2/Velocity Conversion  IU=m/s  OU=ft/s
  Out1 : Outport
  wires:
  Constant12/1 -> Divide1/4
  In2/1 -> Velocity Conversion/1
  In3/1 -> 2-D Lookup Table5/2
  MATLAB Function15/1(y) -> Scope13/1, Product3/1
  Constant10/1 -> Divide1/2
  Product3/1 -> Out1/1, Scope11/1
  Divide1/1 -> Product3/3, Scope10/1
  u/1 -> MATLAB Function15/1(u)
  2-D Lookup Table5/1 -> Product3/2
  In4/1 -> Divide1/1
  In5/1 -> Divide1/3
  Velocity Conversion/1 -> 2-D Lookup Table5/1

== system simulink_flightgear_control_trim_wind_5/Plane/气动系数/Subsystem58/Subsystem60 ==
  In1 : Inport
  In2 : Inport  Port=2
  Radians in : Inport  Port=3
  In4 : Inport  Port=4
  1-D Lookup Table79 : Lookup_n-D  NumberOfTableDimensions=1  BreakpointsForDimension1=P3DAERO.delta_Cl_RL_25(1,:)  Table=P3DAERO.delta_Cl_RL_25(2,:)  InternalRulePriority=Speed  RndMeth=Simplest
  1-D Lookup Table81 : Lookup_n-D  NumberOfTableDimensions=1  BreakpointsForDimension1=P3DAERO.k_delta_RL(1,:)  Table=P3DAERO.k_delta_RL(2,:)  InternalRulePriority=Speed  RndMeth=Simplest
  2-D Lookup Table14 : Lookup_n-D  BreakpointsForDimension1=high1  BreakpointsForDimension2=mach  Table=P3DAERO.delta_Cl_RL_mach  InternalRulePriority=Speed  RndMeth=Simplest
      settings: InputPortMap=u0,u1
  Abs5 : Abs  SaturateOnIntegerOverflow=off
  Constant34 : Constant
  Constant35 : Constant  Value=-1
  Gain7 : Gain  Gain=m2ft
  Product8 : Product  Inputs=4
  Radians to Degrees22 : simulink_extras/Transformations/Radians to Degrees
  Radians to Degrees23 : simulink_extras/Transformations/Radians to Degrees
  Switch6 : Switch  SaturateOnIntegerOverflow=off  InputSameDT=off
  Out1 : Outport
  wires:
  Switch6/1 -> Product8/4
  Constant34/1 -> Switch6/1
  Radians to Degrees23/1 -> Abs5/1
  Radians to Degrees22/1 -> 1-D Lookup Table79/1
  In4/1 -> Switch6/2, Radians to Degrees23/1
  1-D Lookup Table81/1 -> Product8/3
  2-D Lookup Table14/1 -> Product8/1
  Abs5/1 -> 1-D Lookup Table81/1
  Constant35/1 -> Switch6/3
  In2/1 -> 2-D Lookup Table14/2
  1-D Lookup Table79/1 -> Product8/2
  Gain7/1 -> 2-D Lookup Table14/1
  Product8/1 -> Out1/1
  Radians in/1 -> Radians to Degrees22/1
  In1/1 -> Gain7/1

== system simulink_flightgear_control_trim_wind_5/Plane/气动系数/Subsystem58/Subsystem61 ==
  In1 : Inport
  In2 : Inport  Port=2
  Radians in : Inport  Port=3
  Radians in1 : Inport  Port=4
  1-D Lookup Table101 : Lookup_n-D  NumberOfTableDimensions=1  BreakpointsForDimension1=P3DAERO.delata_CN_RU_25(1,:)  Table=P3DAERO.delata_CN_RU_25(2,:)  InternalRulePriority=Speed  RndMeth=Simplest
  1-D Lookup Table102 : Lookup_n-D  NumberOfTableDimensions=1  BreakpointsForDimension1=P3DAERO.k_delta_RU(1,:)  Table=P3DAERO.k_delta_RU(2,:)  InternalRulePriority=Speed  RndMeth=Simplest
  2-D Lookup Table14 : Lookup_n-D  BreakpointsForDimension1=high1  BreakpointsForDimension2=mach  Table=P3DAERO.delata_CN_RU_25_mach  InternalRulePriority=Speed  RndMeth=Simplest
      settings: InputPortMap=u0,u1
  Abs : Abs  SaturateOnIntegerOverflow=off
  Constant32 : Constant
  Constant33 : Constant  Value=-1
  Gain9 : Gain  Gain=m2ft
  Product7 : Product  Inputs=4
  Radians to Degrees20 : simulink_extras/Transformations/Radians to Degrees
  Radians to Degrees21 : simulink_extras/Transformations/Radians to Degrees
  Scope : Scope
  Switch12 : Switch  SaturateOnIntegerOverflow=off  InputSameDT=off
  Out1 : Outport
  wires:
  Abs/1 -> 1-D Lookup Table102/1
  Radians to Degrees21/1 -> Abs/1
  Switch12/1 -> Product7/4
  In1/1 -> Gain9/1
  1-D Lookup Table102/1 -> Product7/3
  Gain9/1 -> 2-D Lookup Table14/1
  Radians to Degrees20/1 -> 1-D Lookup Table101/1
  Constant33/1 -> Switch12/3
  2-D Lookup Table14/1 -> Product7/1
  Constant32/1 -> Switch12/1
  1-D Lookup Table101/1 -> Product7/2
  Radians in1/1 -> Switch12/2, Radians to Degrees21/1
  Product7/1 -> Scope/1, Out1/1
  Radians in/1 -> Radians to Degrees20/1
  In2/1 -> 2-D Lookup Table14/2

== system simulink_flightgear_control_trim_wind_5/Plane/气动系数/Subsystem58/Subsystem62 ==
  note: beta地效修正
  note: 米变英尺
  In1 : Inport
  In2 : Inport  Port=2
  Radians in : Inport  Port=3
  1-D Lookup Table97 : Lookup_n-D  NumberOfTableDimensions=1  BreakpointsForDimension1=P3DAERO.k_ge(1,:)  Table=P3DAERO.k_ge(2,:)  InternalRulePriority=Speed  RndMeth=Simplest
  2-D Lookup Table4 : Lookup_n-D  BreakpointsForDimension1=flap  BreakpointsForDimension2=alpha1  Table=P3DAERO.F_rho_beta  InternalRulePriority=Speed  RndMeth=Simplest
      settings: InputPortMap=u0,u1
  Constant21 : Constant
  Gain14 : Gain  Gain=m2ft
  Product16 : Product
  Radians to Degrees4 : simulink_extras/Transformations/Radians to Degrees
  Saturation4 : Saturate  UpperLimit=14  LowerLimit=0
  Scope31 : Scope
  Scope48 : Scope
  Sum11 : Sum
  Switch5 : Switch  Criteria=u2 > Threshold  Threshold=24  SaturateOnIntegerOverflow=off  InputSameDT=off
  Out1 : Outport
  wires:
  Sum11/1 -> Switch5/3
  Product16/1 -> Sum11/2
  In2/1 -> 2-D Lookup Table4/1
  In1/1 -> Switch5/2, Gain14/1
  Radians to Degrees4/1 -> Saturation4/1
  Radians in/1 -> Radians to Degrees4/1
  Constant21/1 -> Sum11/1, Switch5/1
  2-D Lookup Table4/1 -> Product16/2
  Saturation4/1 -> 2-D Lookup Table4/2
  Gain14/1 -> 1-D Lookup Table97/1
  1-D Lookup Table97/1 -> Scope48/1, Product16/1
  Switch5/1 -> Out1/1, Scope31/1

== system simulink_flightgear_control_trim_wind_5/Plane/气动系数/Subsystem58/Subsystem63 ==
  In1 : Inport
  In2 : Inport  Port=2
  Radians in : Inport  Port=3
  Radians in1 : Inport  Port=4
  In5 : Inport  Port=5
  2-D Lookup Table : Lookup_n-D  BreakpointsForDimension1=flap  BreakpointsForDimension2=alpha  Table=P3DAERO.dot_Cl_dot_beta_lowspeed  InternalRulePriority=Speed  RndMeth=Simplest
      settings: InputPortMap=u0,u1
  2-D Lookup Table1 : Lookup_n-D  BreakpointsForDimension1=mach2  BreakpointsForDimension2=alpha  Table=P3DAERO.dot_Cl_dot_beta_highspeed  InternalRulePriority=Speed  RndMeth=Simplest
      settings: InputPortMap=u0,u1
  2-D Lookup Table2 : Lookup_n-D  BreakpointsForDimension1=flap  BreakpointsForDimension2=beta  Table=P3DAERO.dot_Cl_beta  InternalRulePriority=Speed  RndMeth=Simplest
      settings: InputPortMap=u0,u1
  2-D Lookup Table3 : Lookup_n-D  BreakpointsForDimension1=high1  BreakpointsForDimension2=mach  Table=P3DAERO.dot_Cl_aeroelastic  InternalRulePriority=Speed  RndMeth=Simplest
      settings: InputPortMap=u0,u1
  Gain4 : Gain  Gain=m2ft
  Product2 : Product  Inputs=3
  Radians to Degrees : simulink_extras/Transformations/Radians to Degrees
  Radians to Degrees2 : simulink_extras/Transformations/Radians to Degrees
  Saturation1 : Saturate  UpperLimit=1  LowerLimit=0
  Scope{2,7..9} (4 alike) : Scope
  Switch2 : Switch  Criteria=u2 ~= 0  Threshold=0.35  SaturateOnIntegerOverflow=off  InputSameDT=off
  Out1 : Outport
  wires:
  2-D Lookup Table1/1 -> Switch2/3
  Switch2/1 -> Product2/1, Scope8/1
  In2/1 -> 2-D Lookup Table/1, 2-D Lookup Table2/1
  2-D Lookup Table3/1 -> Scope2/1, Product2/3
  Radians to Degrees/1 -> 2-D Lookup Table/2, 2-D Lookup Table1/2
  2-D Lookup Table/1 -> Switch2/1
  2-D Lookup Table2/1 -> Saturation1/1, Scope9/1
  In1/1 -> 2-D Lookup Table1/1, Switch2/2, 2-D Lookup Table3/2
  Radians in1/1 -> Radians to Degrees2/1
  Radians to Degrees2/1 -> 2-D Lookup Table2/2
  Gain4/1 -> 2-D Lookup Table3/1
  Radians in/1 -> Radians to Degrees/1
  In5/1 -> Gain4/1
  Saturation1/1 -> Product2/2
  Product2/1 -> Scope7/1, Out1/1

== system simulink_flightgear_control_trim_wind_5/Plane/气动系数/Subsystem58/Subsystem64 ==
  note: 滚转角速度
  note: 速度ft/s
  In1 : Inport
  Radians in : Inport  Port=2
  In3 : Inport  Port=3
  In4 : Inport  Port=4
  In5 : Inport  Port=5
  In6 : Inport  Port=6
  2-D Lookup Table5 : Lookup_n-D  BreakpointsForDimension1=flap  BreakpointsForDimension2=alpha  Table=P3DAERO.doe_Cl_dot_p  InternalRulePriority=Speed  RndMeth=Simplest
      settings: InputPortMap=u0,u1
  2-D Lookup Table6 : Lookup_n-D  BreakpointsForDimension1=high1  BreakpointsForDimension2=mach  Table=P3DAERO.doe_Cl_dot_p_mach  InternalRulePriority=Speed  RndMeth=Simplest
      settings: InputPortMap=u0,u1
  Constant10 : Constant  Value=2
  Constant12 : Constant  Value=195.7
  Divide1 : Product  Inputs=**//
  Gain9 : Gain  Gain=m2ft
  Product3 : Product  Inputs=3
  Radians to Degrees5 : simulink_extras/Transformations/Radians to Degrees
  Scope : Scope
  Scope1 : Scope
  Out1 : Outport
  wires:
  In4/1 -> 2-D Lookup Table6/2
  Divide1/1 -> Product3/3
  2-D Lookup Table5/1 -> Product3/1
  Constant12/1 -> Divide1/2
  Constant10/1 -> Divide1/4
  Radians to Degrees5/1 -> 2-D Lookup Table5/2
  In1/1 -> 2-D Lookup Table5/1
  2-D Lookup Table6/1 -> Product3/2
  In5/1 -> Scope1/1, Divide1/1
  In3/1 -> Gain9/1
  Radians in/1 -> Radians to Degrees5/1
  In6/1 -> Divide1/3
  Product3/1 -> Scope/1, Out1/1
  Gain9/1 -> 2-D Lookup Table6/1

== system simulink_flightgear_control_trim_wind_5/Plane/气动系数/Subsystem58/Subsystem65 ==
  note: 速度ft/s
  note: 偏航角速度
  In1 : Inport
  Radians in : Inport  Port=2
  In3 : Inport  Port=3
  In4 : Inport  Port=4
  In5 : Inport  Port=5
  In6 : Inport  Port=6
  2-D Lookup Table7 : Lookup_n-D  BreakpointsForDimension1=flap  BreakpointsForDimension2=alpha  Table=P3DAERO.doe_Cl_dot_r  InternalRulePriority=Speed  RndMeth=Simplest
      settings: InputPortMap=u0,u1
  2-D Lookup Table8 : Lookup_n-D  BreakpointsForDimension1=high1  BreakpointsForDimension2=mach  Table=P3DAERO.doe_Cl_dot_r_mach  InternalRulePriority=Speed  RndMeth=Simplest
      settings: InputPortMap=u0,u1
  Constant7 : Constant  Value=2
  Constant8 : Constant  Value=195.7
  Divide2 : Product  Inputs=**//
  Gain : Gain
  Gain9 : Gain  Gain=m2ft
  Product2 : Product  Inputs=3
  Radians to Degrees6 : simulink_extras/Transformations/Radians to Degrees
  Scope{,1..3} (4 alike) : Scope
  Out1 : Outport
  wires:
  Constant7/1 -> Divide2/4
  In4/1 -> 2-D Lookup Table8/2
  Radians to Degrees6/1 -> 2-D Lookup Table7/2
  2-D Lookup Table7/1 -> Scope2/1, Product2/1
  Divide2/1 -> Product2/3
  Constant8/1 -> Divide2/2
  2-D Lookup Table8/1 -> Product2/2
  In5/1 -> Scope1/1, Divide2/1
  Radians in/1 -> Radians to Degrees6/1
  In1/1 -> 2-D Lookup Table7/1
  In3/1 -> Gain9/1
  Product2/1 -> Scope3/1, Gain/1
  Gain/1 -> Scope/1, Out1/1
  In6/1 -> Divide2/3
  Gain9/1 -> 2-D Lookup Table8/1

== system simulink_flightgear_control_trim_wind_5/Plane/气动系数/Subsystem58/Subsystem66 ==
  note: dot_CL_dot_delta
  In1 : Inport
  In2 : Inport  Port=2
  In3 : Inport  Port=3
  Radians in : Inport  Port=4
  2-D Lookup Table9 : Lookup_n-D  BreakpointsForDimension1=high1  BreakpointsForDimension2=mach  Table=P3DAERO.dot_CL_dot_delta  InternalRulePriority=Speed  RndMeth=Simplest
      settings: InputPortMap=u0,u1
  Product5 : Product  Inputs=3
  Radians to Degrees3 : simulink_extras/Transformations/Radians to Degrees
  Scope17 : Scope
  Velocity Conversion : aerolibconvert2/Velocity Conversion  IU=m/s  OU=ft/s
  Out1 : Outport
  wires:
  Radians in/1 -> Radians to Degrees3/1
  In2/1 -> Velocity Conversion/1
  Radians to Degrees3/1 -> Product5/3
  Product5/1 -> Out1/1, Scope17/1
  2-D Lookup Table9/1 -> Product5/2
  In1/1 -> Product5/1
  In3/1 -> 2-D Lookup Table9/2
  Velocity Conversion/1 -> 2-D Lookup Table9/1

== system simulink_flightgear_control_trim_wind_5/Plane/气动系数/Subsystem58/Subsystem67 ==
  note: 襟翼角度
  In1 : Inport
  In2 : Inport  Port=2
  Radians in : Inport  Port=3
  In4 : Inport  Port=4
  1-D Lookup Table91 : Lookup_n-D  NumberOfTableDimensions=1  BreakpointsForDimension1=P3DAERO.mach_gear(1,:)  Table=P3DAERO.mach_gear(2,:)  InternalRulePriority=Speed  RndMeth=Simplest
  2-D Lookup Table17 : Lookup_n-D  BreakpointsForDimension1=flap  BreakpointsForDimension2=alpha  Table=P3DAERO.deltaCL_gear  InternalRulePriority=Speed  RndMeth=Simplest
      settings: InputPortMap=u0,u1
  Gain : Gain
  Gain1 : Gain  Gain=-1
  Product15 : Product  Inputs=3
  Radians to Degrees2 : simulink_extras/Transformations/Radians to Degrees
  Scope47 : Scope
  Out1 : Outport
  wires:
  Radians in/1 -> Radians to Degrees2/1
  In1/1 -> Product15/1
  In4/1 -> 1-D Lookup Table91/1
  2-D Lookup Table17/1 -> Product15/2
  1-D Lookup Table91/1 -> Product15/3
  Radians to Degrees2/1 -> 2-D Lookup Table17/2
  In2/1 -> 2-D Lookup Table17/1
  Product15/1 -> Gain/1, Scope47/1
  Gain/1 -> Out1/1
